simulink model "BlocoHidraulicoLAC_OpenLoop"  (R2026a)
settings: Solver=ode15s  StopTime=5  MaxStep=1e-4
undefined symbols (not defined in the file or in its folder): sigbuilder_block
(part 1 of 2)
settings Model: Creator=uidq5744  LastModifiedBy=uidq5744

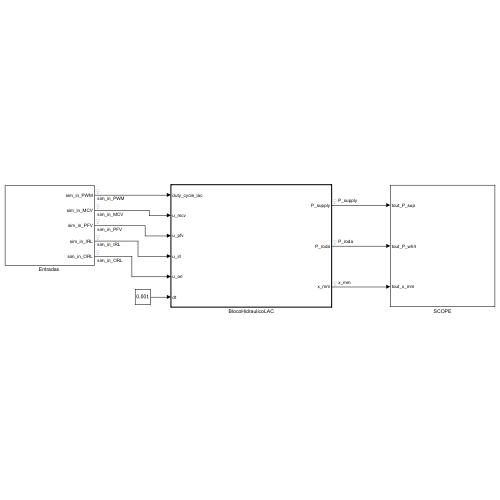
[thumbnail: Simulink's stored preview of the top-level diagram]
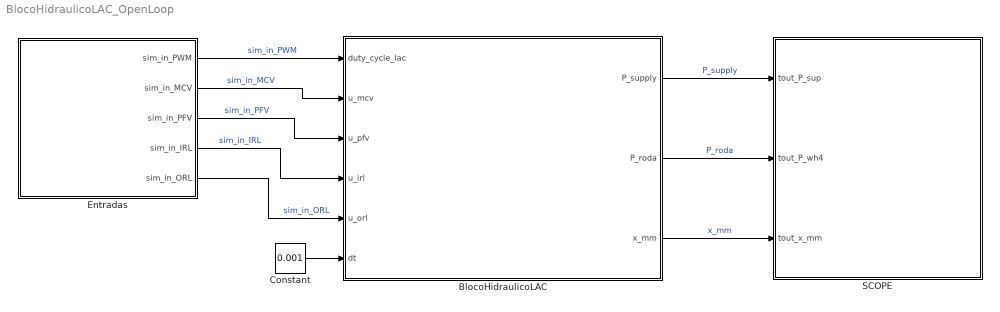
== system BlocoHidraulicoLAC_OpenLoop ==
  " BlocoHidraulicoLAC " : MATLAB Function  TreatAsAtomicUnit=on
  Constant : Constant  Value=0.001
  "Entradas " : Subsystem
  SCOPE : Subsystem
  wires:
  "Entradas "/3(sim_in_PFV) -> " BlocoHidraulicoLAC "/3(u_pfv)  "sim_in_PFV"
  "Entradas "/4(sim_in_IRL) -> " BlocoHidraulicoLAC "/4(u_irl)  "sim_in_IRL"
  "Entradas "/2(sim_in_MCV) -> " BlocoHidraulicoLAC "/2(u_mcv)  "sim_in_MCV"
  "Entradas "/1(sim_in_PWM) -> " BlocoHidraulicoLAC "/1(duty_cycle_lac)  "sim_in_PWM"
  "Entradas "/5(sim_in_ORL) -> " BlocoHidraulicoLAC "/5(u_orl)  "sim_in_ORL"
  " BlocoHidraulicoLAC "/1(P_supply) -> SCOPE/1(tout_P_sup)  "P_supply"
  " BlocoHidraulicoLAC "/2(P_roda) -> SCOPE/2(tout_P_wh4)  "P_roda"
  Constant/1 -> " BlocoHidraulicoLAC "/6(dt)
  " BlocoHidraulicoLAC "/3(x_mm) -> SCOPE/3(tout_x_mm)  "x_mm"

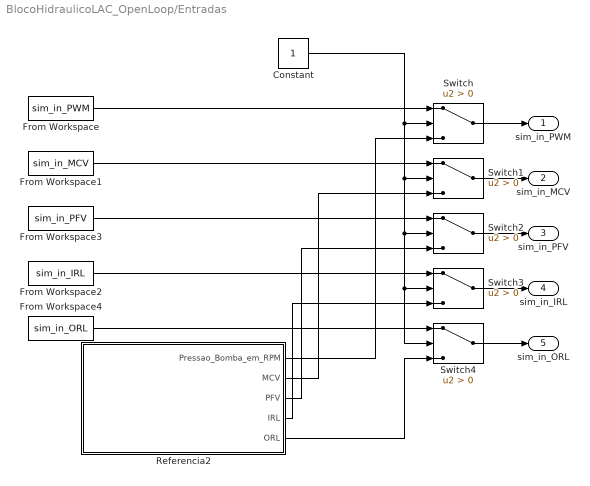
== system BlocoHidraulicoLAC_OpenLoop/Entradas  ==
  Constant : Constant
  From Workspace : FromWorkspace  VariableName=sim_in_PWM
  From Workspace1 : FromWorkspace  VariableName=sim_in_MCV
  From Workspace2 : FromWorkspace  VariableName=sim_in_IRL
  From Workspace3 : FromWorkspace  VariableName=sim_in_PFV
  From Workspace4 : FromWorkspace  VariableName=sim_in_ORL
  Referencia2 : Subsystem  Tag=STV Subsys  LoadFcn=sigbuilder_block('load',[316.5 -63 1440 720 ]);  StartFcn=sigbuilder_block('start');  StopFcn=sigbuilder_block('stop');  ClipboardFcn=sigbuilder_block('clipboard');  mask(Sigbuilder block){tuvar=[0:10]}
      mask help: Simulink:masks:SigbuilderBlock_MD
      mask init:
      | if ~strcmp(get_param(bdroot(gcbh),'SimulationStatus'),'stopped') tuvar = sigbuilder_block('maskInit'); end
      settings: CopyFcn=sigbuilder_block('copy');  DeleteFcn=sigbuilder_block('delete');  ModelCloseFcn=sigbuilder_block('modelClose');  PreSaveFcn=sigbuilder_block('preSave');  PauseFcn=sigbuilder_block('pause');  ContinueFcn=sigbuilder_block('continue');  NameChangeFcn=sigbuilder_block('namechange');  OpenFcn=sigbuilder_block('open',[323.25 1076.25 805.5 485.25 ]);  CloseFcn=sigbuilder_block('close');
      mask Display: plot(0, 0, 100, 100,[2, 2, 32, 32, 2], [68, 8, 8, 68, 68],[32, 2], [38, 38], [32, 19, 2],[53, 60, 44], [32, 17, 17, 2],[16, 16, 31, 31]);txt = getActiveGroup(gcbh);text(2, 100, txt,'verticalAlignment', 'top');
  Switch{,1..4} (5 alike) : Switch  Criteria=u2 > Threshold  SaturateOnIntegerOverflow=off  InputSameDT=off
  sim_in_PWM : Outport
  sim_in_MCV : Outport  Port=2
  sim_in_PFV : Outport  Port=3
  sim_in_IRL : Outport  Port=4
  sim_in_ORL : Outport  Port=5
  wires:
  Referencia2/1(Pressao_Bomba_em_RPM) -> Switch/3
  Referencia2/2(MCV) -> Switch1/3
  Referencia2/4(IRL) -> Switch3/3
  Referencia2/3(PFV) -> Switch2/3
  Referencia2/5(ORL) -> Switch4/3
  From Workspace/1 -> Switch/1
  Switch/1 -> sim_in_PWM/1
  Switch1/1 -> sim_in_MCV/1
  Switch2/1 -> sim_in_PFV/1
  Switch3/1 -> sim_in_IRL/1
  Switch4/1 -> sim_in_ORL/1
  From Workspace1/1 -> Switch1/1
  From Workspace4/1 -> Switch4/1
  From Workspace2/1 -> Switch3/1
  From Workspace3/1 -> Switch2/1
  Constant/1 -> Switch/2, Switch1/2, Switch2/2, Switch3/2, Switch4/2

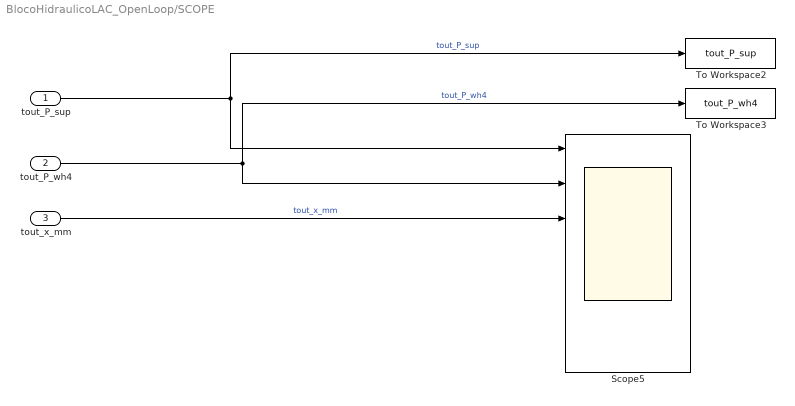
== system BlocoHidraulicoLAC_OpenLoop/SCOPE ==
  tout_P_sup : Inport
  tout_P_wh4 : Inport  Port=2
  tout_x_mm : Inport  Port=3
  Scope5 : Scope  NumInputPorts=7
      settings: ActiveDisplayYMinimum=-5.7644121130531885E+294  ActiveDisplayYMaximum=5.18797090174787E+295  DataLoggingVariableName=ScopeData6
  To Workspace2 : ToWorkspace  VariableName=tout_P_sup  SaveFormat=Timeseries  SampleTime=-1
  To Workspace3 : ToWorkspace  VariableName=tout_P_wh4  SaveFormat=Timeseries  SampleTime=-1
  wires:
  tout_P_sup/1 -> Scope5/1, To Workspace2/1  "tout_P_sup"
  tout_P_wh4/1 -> Scope5/2, To Workspace3/1  "tout_P_wh4"
  tout_x_mm/1 -> Scope5/3  "tout_x_mm"

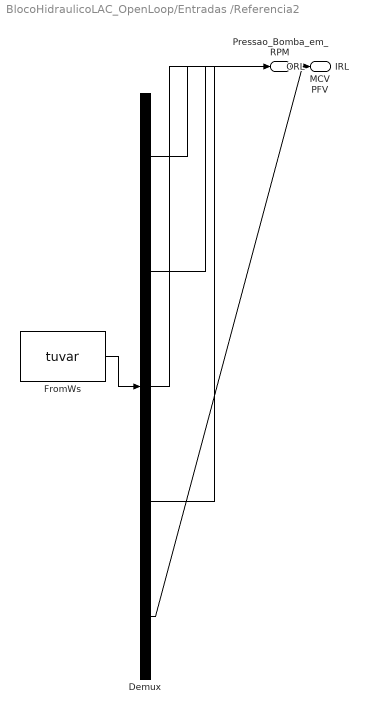
== system BlocoHidraulicoLAC_OpenLoop/Entradas /Referencia2 ==
  Demux : Demux  Tag=STV Demux  Outputs=5
      settings: DisplayOption=none
  FromWs : FromWorkspace  Tag=STV FromWs  VariableName=tuvar
      SigBuilderData=|
      | common.afterFinalStr = 'Extrapolate'
      | common.sampleTime = 0
      | dataSet.timeRange = [0 50]
      | dataSet.name = 'Group 1'
      | sbobj.Groups.Name = 'Group 1'
      | sbobj.Groups.Signals(1).Name = 'Pressao_Bomba_em_RPM'
      | sbobj.Groups.Signals(1).XData = [0 1 1 1.015 1.015 5.11 5.11 5.465 5.465 48.3 48.3 50]
      | sbobj.Groups.Signals(1).YData = [0 0 50 50 0 0 50 50 0 0 30 85]
      | sbobj.Groups.Signals(2).Name = 'MCV'
      | sbobj.Groups.Signals(2).XData = [0 1 1 1.045 1.045 5.34 5.34 5.775 5.775 50]
      | sbobj.Groups.Signals(2).YData = [0 0 1 1 0 0 1 1 0 0]
      | sbobj.Groups.Signals(3).Name = 'PFV'
      | sbobj.Groups.Signals(3).XData = [0 1 1 1.045 1.045 5.45 5.45 6.075 6.075 50]
      | sbobj.Groups.Signals(3).YData = [0 0 1 1 0 0 1 1 0 0]
      | sbobj.Groups.Signals(4).Name = 'IRL'
      | sbobj.Groups.Signals(4).XData = [0 1 1 1.045 1.045 5.55 5.55 6.025 6.025 50]
      | sbobj.Groups.Signals(4).YData = [0 0 1 1 0 0 1 1 0 0]
      | sbobj.Groups.Signals(5).Name = 'ORL'
      | sbobj.Groups.Signals(5).XData = [0 3 3 4 4 15 20 50]
      | sbobj.Groups.Signals(5).YData = [0 0 1 1 0 0 0 0]
      | sbobj.Groups.TimeRange = [0 50]
  Pressao_Bomba_em_RPM : Outport  Tag=STV Outport
  MCV : Outport  Tag=STV Outport  Port=2
  PFV : Outport  Tag=STV Outport  Port=3
  IRL : Outport  Tag=STV Outport  Port=4
  ORL : Outport  Tag=STV Outport  Port=5
  wires:
  Demux/1 -> Pressao_Bomba_em_RPM/1
  FromWs/1 -> Demux/1
  Demux/2 -> MCV/1
  Demux/3 -> PFV/1
  Demux/4 -> IRL/1
  Demux/5 -> ORL/1
